simulink model "PID"  (R2023a)
settings: Solver=VariableStepAuto  StartTime=0.0  StopTime=10.0  RelTol=1e-3
values from neighbouring files (symbols this model uses):
  PID_Kaw = 0    [load_pid.m]
  PID_Kd = 0    [load_pid.m]
  PID_Ki = 0    [load_pid.m]
  PID_Kp = 0    [load_pid.m]
  PID_Tf = 0.005    [load_pid.m]
  Ts_ctrl = J.Ts_ctrl    [load_pid.m]
undefined symbols (not defined in the file or in its folder): DiscIntNeverNeededParam, Tdref_ay_bp_ms2, Tdref_table, Tdref_v_bp_ms
settings Model: Creator=Tan_Tram  LastModifiedBy=Tan_Tram

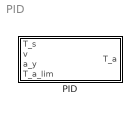
== system PID ==
  PID : Subsystem

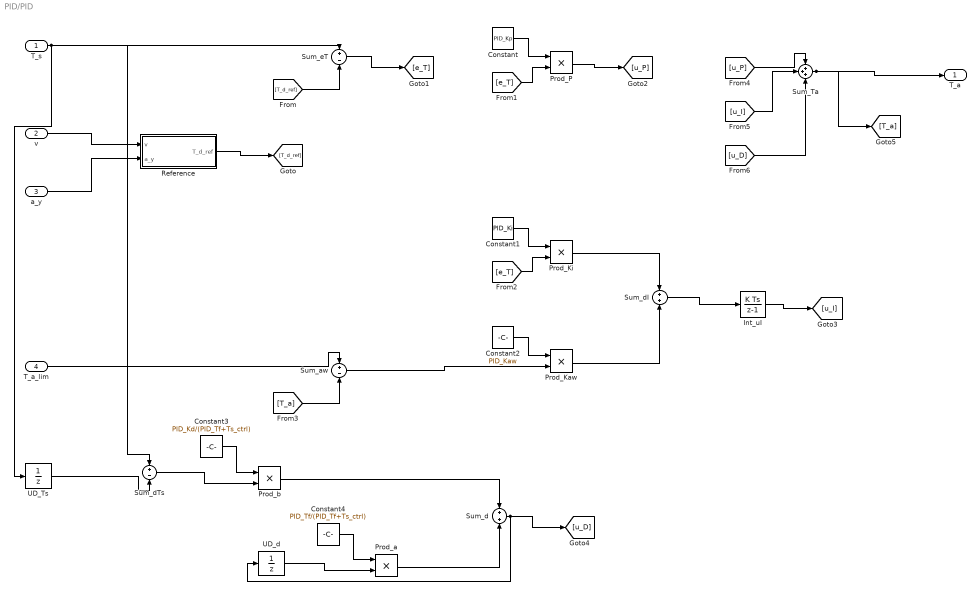
== system PID/PID ==
  T_s : Inport
  v : Inport  Port=2
  a_y : Inport  Port=3
  T_a_lim : Inport  Port=4
  Constant : Constant  Value=PID_Kp
  Constant1 : Constant  Value=PID_Ki
  Constant2 : Constant  Value=PID_Kaw
  Constant3 : Constant  Value=PID_Kd/(PID_Tf+Ts_ctrl)
  Constant4 : Constant  Value=PID_Tf/(PID_Tf+Ts_ctrl)
  Int_uI : DiscreteIntegrator  gainval=1  SampleTime=Ts_ctrl  ICPrevOutput=DiscIntNeverNeededParam  ICPrevScaledInput=DiscIntNeverNeededParam
  Prod_Kaw : Product  Inputs=**
  Prod_Ki : Product  Inputs=**
  Prod_P : Product  Inputs=**
  Prod_a : Product  Inputs=**
  Prod_b : Product  Inputs=**
  Reference : Subsystem
  Sum_Ta : Sum  Inputs=+++
  Sum_aw : Sum  Inputs=+-
  Sum_d : Sum
  Sum_dI : Sum
  Sum_dTs : Sum  Inputs=+-
  Sum_eT : Sum  Inputs=+-
  UD_Ts : UnitDelay  SampleTime=Ts_ctrl  HasFrameUpgradeWarning=on
  UD_d : UnitDelay  SampleTime=Ts_ctrl  HasFrameUpgradeWarning=on
  T_a : Outport
  wires:
  v/1 -> Reference/1(v)
  a_y/1 -> Reference/2(a_y)
  Reference/1(T_d_ref) -> [T_d_ref]
  T_s/1 -> Sum_eT/1, UD_Ts/1, Sum_dTs/1
  [T_d_ref] -> Sum_eT/2
  Sum_eT/1 -> [e_T]
  Constant/1 -> Prod_P/1
  [e_T] -> Prod_P/2
  Prod_P/1 -> [u_P]
  Constant1/1 -> Prod_Ki/1
  [e_T] -> Prod_Ki/2
  T_a_lim/1 -> Sum_aw/1
  [T_a] -> Sum_aw/2
  Constant2/1 -> Prod_Kaw/1
  Sum_aw/1 -> Prod_Kaw/2
  Prod_Ki/1 -> Sum_dI/1
  Prod_Kaw/1 -> Sum_dI/2
  Sum_dI/1 -> Int_uI/1
  Int_uI/1 -> [u_I]
  UD_Ts/1 -> Sum_dTs/2
  Constant3/1 -> Prod_b/1
  Sum_dTs/1 -> Prod_b/2
  Constant4/1 -> Prod_a/1
  UD_d/1 -> Prod_a/2
  Prod_b/1 -> Sum_d/1
  Prod_a/1 -> Sum_d/2
  Sum_d/1 -> UD_d/1, [u_D]
  [u_P] -> Sum_Ta/1
  [u_I] -> Sum_Ta/2
  [u_D] -> Sum_Ta/3
  Sum_Ta/1 -> T_a/1, [T_a]

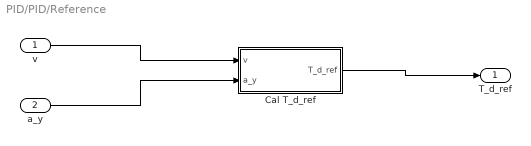
== system PID/PID/Reference ==
  v : Inport
  a_y : Inport  Port=2
  Cal T_d_ref : Subsystem
  T_d_ref : Outport
  wires:
  Cal T_d_ref/1(T_d_ref) -> T_d_ref/1
  a_y/1 -> Cal T_d_ref/2(a_y)
  v/1 -> Cal T_d_ref/1(v)

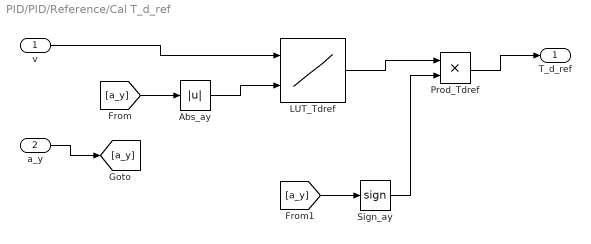
== system PID/PID/Reference/Cal T_d_ref ==
  v : Inport
  a_y : Inport  Port=2
  Abs_ay : Abs  SaturateOnIntegerOverflow=off
  LUT_Tdref : Lookup_n-D  BreakpointsForDimension1=Tdref_v_bp_ms  BreakpointsForDimension2=Tdref_ay_bp_ms2  Table=Tdref_table  ExtrapMethod=Clip  InternalRulePriority=Speed  RndMeth=Simplest
      settings: InputPortMap=u0,u1
  Prod_Tdref : Product  Inputs=**
  Sign_ay : Signum
  T_d_ref : Outport
  wires:
  Prod_Tdref/1 -> T_d_ref/1
  Sign_ay/1 -> Prod_Tdref/2
  LUT_Tdref/1 -> Prod_Tdref/1
  [a_y] -> Sign_ay/1
  Abs_ay/1 -> LUT_Tdref/2
  [a_y] -> Abs_ay/1
  v/1 -> LUT_Tdref/1
  a_y/1 -> [a_y]
